simulink model "FullAssembly"  (R2025b)
settings: Solver=ode23t  StartTime=0.0  StopTime=16  MaxStep=0.25  RelTol=1e-3
model workspace: external: MATLAB File E:\Apps\AutodeskInventor\University\MCT333_Design_of_Mechatronics_Systems_1\matlab_simulation\FullAssembly_DataFile.m (data not in the file)
undefined symbols (not defined in the file or in its folder): smiData, X, Y, Z
libraries: sm_lib x111, Contact_Forces_Lib x19, nesl_utility x6, SignalEditorBlockLib x1
(part 4 of 4)

== stateflow chart FullAssembly/Chart ==
  state Initialize
    entry:
    magazine_cmd = 0;
    piston_cmd = 0;
    x_target = 0;
    y_target = 0;
    z_target = 0;
    gripper_cmd = 0;
  state RotateMagazine
    entry:
    magazine_cmd = 1;
  state ExtendPiston
    entry:
    magazine_cmd = 0;
    piston_cmd = 0.08;
  state ProductDetected
    entry:
    magazine_cmd = 0;
  state RetractPiston
    entry:
    piston_cmd = 0;
  state WaitForSorting
    entry:
    piston_cmd = 0;
  state RobotOperation
    state ReturnDangerHeight
      entry:
      z_target = safe_z;
    state MoveAbovePickup
      entry:
      z_target = safe_z;
      x_target = pickup_x;
      y_target = pickup_y;
      robot_done=false;
      robot_busy = true;
    state LowerSuctionCup
      entry:
      z_target = pickup_z;
    state ActivateVacuum
      entry:
      vacuum_cmd = 1;
    state LiftProduct
      entry:
      z_target = safe_z;
    state MoveAboveDestination
      entry:
      x_target = destination_x;
      y_target = destination_y;
    state LowerToPlace
      entry:
      z_target = destination_z;
    state DeactivateVacuum
    state ReturnSafeHeight
      entry:
      z_target = safe_z;
    state RobotCompleted
      entry:
      robot_done = true;
      robot_busy = false;
      robot_operation_complete = true;
    (default) -> ReturnDangerHeight
    ReturnDangerHeight -> MoveAbovePickup : [abs(z_pos-safe_z) < position_tolerance]
    MoveAbovePickup -> LowerSuctionCup : [abs(x_pos-pickup_x)<position_tolerance && ...
        |  abs(y_pos-pickup_y)<position_tolerance && ...
        |  abs(z_pos-safe_z)<position_tolerance]
    LowerSuctionCup -> ActivateVacuum : [abs(z_pos-pickup_z)<position_tolerance]
    ActivateVacuum -> LiftProduct : [vacuum_confirmed == 1]
    LiftProduct -> MoveAboveDestination : [abs(z_pos-safe_z)<position_tolerance]
    MoveAboveDestination -> LowerToPlace : [abs(x_pos-destination_x)<position_tolerance && ...
        |  abs(y_pos-destination_y)<position_tolerance]
    LowerToPlace -> DeactivateVacuum : [abs(z_pos-destination_z)<position_tolerance]
    DeactivateVacuum -> ReturnSafeHeight : [vacuum_confirmed == 0]
    ReturnSafeHeight -> RobotCompleted : [abs(z_pos-safe_z)<position_tolerance]
  state ClassifyProduct
    entry:
    piston_cmd = 0;
  state DecideDestination
    entry:
    product_code = 2*inductive_sensor + laser_upper + 1;
  state FindStorage
    entry:
    destination_slot = uint8(0);
    destination_type = uint8(0);
    if product_code == 1
    % NON-METAL LID
    for i = 5:8
    if final_status(i) == 1
    destination_slot = uint8(i);
    destination_type = uint8(2);
    break;
    end
    end
    elseif product_code == 2
    % NON-METAL BASE
    for i = 5:8
    if final_status(i) == 0
    destination_slot = uint8(i);
    destination_type = uint8(2);
    break;
    end
    end
    elseif product_code == 3
    % METAL LID
    for i = 1:4
    if final_status(i) == 1
    destination_slot = uint8(i);
    destination_type = uint8(2);
    break;
    end
    end
    elseif product_code == 4
    % METAL BASE
    for i = 1:4
    if final_status(i) == 0
    destination_slot = uint8(i);
    destination_type = uint8(2);
    break;
    end
    end
    end
    % If a lid has no matching base, use temporary storage
    if destination_slot == 0 && (product_code == 1 || product_code == 3)
    for i = 1:8
    if temp_status(i) == 0
    destination_slot = uint8(i);
    destination_type = uint8(1);
    break;
    end
    end
    end
  state PrepareRobotMove
    entry:
    robot_mode = uint8(1);
    robot_operation_complete = false;
    pickup_x = sorting_x;
    pickup_y = sorting_y;
    if destination_type == 1
    destination_x = temp_x(destination_slot);
    destination_y = temp_y(destination_slot);
    elseif destination_type == 2
    destination_x = final_x(destination_slot);
    destination_y = final_y(destination_slot);
    end
  state UpdateStorage
    entry:
    if destination_type == 1
    % Product placed in temporary storage
    if product_code == 1
    temp_status(destination_slot) = uint8(1);
    elseif product_code == 3
    temp_status(destination_slot) = uint8(2);
    end
    elseif destination_type == 2
    % Product placed in final storage
    if product_code == 2 || product_code == 4
    final_status(destination_slot) = uint8(1);
    else
    final_status(destination_slot) = uint8(2);
    assembled_count = assembled_count + uint8(1);
    end
    end
  state CheckWaitingLid
    entry:
    retrieve_required = false;
    retrieve_slot = uint8(0);
    retrieve_final_slot = uint8(0);
    if product_code == 4
    % Metal base was placed
    for i = 1:8
    if temp_status(i) == 2
    retrieve_required = true;
    retrieve_slot = uint8(i);
    retrieve_final_slot = destination_slot;
    break;
    end
    end
    elseif product_code == 2
    % Non-metal base was placed
    for i = 1:8
    if temp_status(i) == 1
    retrieve_required = true;
    retrieve_slot = uint8(i);
    retrieve_final_slot = destination_slot;
    break;
    end
    end
    end
  state PrepareLidRetrieval
    entry:
    robot_mode = uint8(2);
    robot_operation_complete = false;
    pickup_x = temp_x(retrieve_slot);
    pickup_y = temp_y(retrieve_slot);
    destination_x = final_x(retrieve_final_slot);
    destination_y = final_y(retrieve_final_slot);
  state CompleteAssembly
    entry:
    temp_status(retrieve_slot) = uint8(0);
    final_status(retrieve_final_slot) = uint8(2);
    assembled_count = assembled_count + uint8(1);
  state Finished
    entry:
    magazine_cmd = 0;
    piston_cmd = 0;
    gripper_cmd = 0;
  state NextCycle
  Initialize -> ProductDetected [order 2] : [magazine_IR == 1]
  (default) -> Initialize
  PrepareRobotMove -> RobotOperation
  PrepareLidRetrieval -> RobotOperation
  Initialize -> RotateMagazine [order 1] : [magazine_IR == 0]
  ProductDetected -> ExtendPiston
  ExtendPiston -> RetractPiston : [piston_pos >= 0.079]
  RotateMagazine -> ProductDetected : [magazine_IR == 1]
  NextCycle -> RotateMagazine [order 2] : [assembled_count < 8 && magazine_IR == 0]
  RetractPiston -> WaitForSorting : [piston_pos <= 0.001]
  WaitForSorting -> ClassifyProduct : [station_contact == 1]
  ClassifyProduct -> DecideDestination : [laser_lower == 1]
  DecideDestination -> FindStorage
  FindStorage -> PrepareRobotMove : [destination_slot > 0]
  RobotOperation -> UpdateStorage [order 1] : [robot_operation_complete == true && robot_mode == 1]
  CheckWaitingLid -> PrepareLidRetrieval [order 2] : [retrieve_required == true]
  UpdateStorage -> CheckWaitingLid
  CheckWaitingLid -> NextCycle [order 1] : [retrieve_required == false]
  RobotOperation -> CompleteAssembly [order 2] : [robot_operation_complete == true && robot_mode == 2]
  CompleteAssembly -> NextCycle
  NextCycle -> Finished [order 1] : [assembled_count >= 8]
  data: magazine_cmd output double; z_target output double; y_target output double; x_target output double; piston_cmd output double; gripper_cmd output double; magazine_IR input boolean; piston_pos input double size=1; product_code output double; station_contact input boolean; laser_upper input boolean; laser_lower input boolean; inductive_sensor input boolean; final_status local uint8 size=[1 8] =zeros(1,8,'uint8'); temp_status local uint8 size=[1 8] =zeros(1,8,'uint8'); assembled_count local uint8 size=1 =0; destination_slot local uint8 size=1 =0; destination_type local uint8 size=1 =0; i local double size=1 =0; retrieve_slot local uint8 =0; retrieve_final_slot local uint8 =0; retrieve_required local boolean =false; placed_product input boolean; x_pos input double; y_pos input double; z_pos input double; vacuum_confirmed input boolean; vacuum_cmd output double =0; pickup_x local double =0; pickup_y local double =0; pickup_z local double =0; destination_x local double =0; destination_y local double =0; destination_z local double =0; safe_z local double =0; position_tolerance local double =0.002; robot_done local boolean =false; robot_mode local uint8 =0; robot_busy local boolean =false; robot_request local boolean =false; final_x local double size=[1 8] =zeros(1,8); sorting_x local double size=1 =0; final_y local double size=[1 8] =zeros(1,8); final_z local double size=[1 8] =zeros(1,8); temp_x local double size=[1 8] =zeros(1,8); temp_y local double size=[1 8] =zeros(1,8); sorting_y local double size=1 =0; robot_operation_complete local boolean =false
